simulink model "CACC_konvoy"  (R2026a)
settings: Solver=ode4  StopTime=T_stop  FixedStep=dt
values from neighbouring files (symbols this model uses):
  d0 = 5    [CACC_yonetim.m]
  dt = 0.01    [CACC_yonetim.m]
  ff_u = 1    [CACC_yonetim.m]
  h = 0.6    [CACC_yonetim.m]
  Kd = 0.8    [CACC_yonetim.m]
  Kf = Kf_cacc    (= 0.8)    [CACC_yonetim.m]
  Kp = 0.4    [CACC_yonetim.m]
  L = 4.5    [CACC_yonetim.m]
  p0 = -(1:N) * (d_ss + L)    [CACC_yonetim.m]
  tau = 0.5    [CACC_yonetim.m]
  tauc_max = max(tauc_profil(:, 2)) + dt    [CACC_yonetim.m]
  u_max = 3    [CACC_yonetim.m]
  u_min = -5    [CACC_yonetim.m]
  v0 = 15    [CACC_yonetim.m]
settings Model: Creator=furka  LastModifiedBy=furka

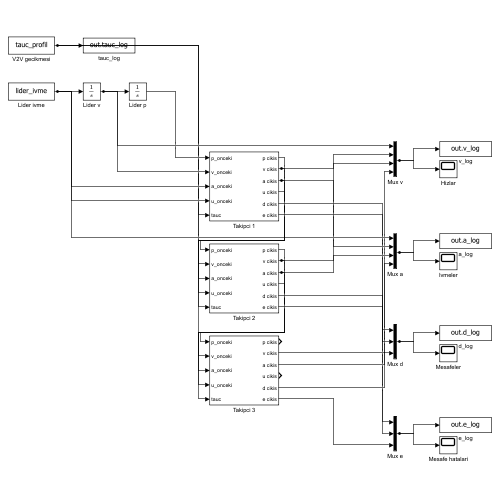
[thumbnail: Simulink's stored preview of the top-level diagram]
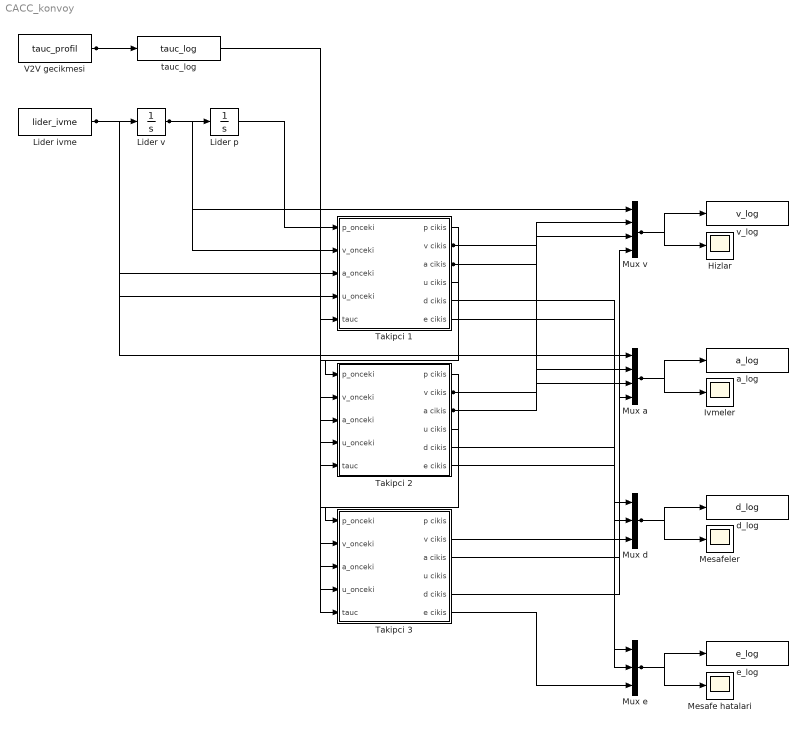
== system CACC_konvoy ==
  Hizlar : Scope
  Ivmeler : Scope
  Lider ivme : FromWorkspace  VariableName=lider_ivme  OutputAfterFinalValue=Holding final value
  Lider p : Integrator
  Lider v : Integrator  InitialCondition=v0
  Mesafe hatalari : Scope
  Mesafeler : Scope
  Mux a : Mux
  Mux d : Mux  Inputs=3
  Mux e : Mux  Inputs=3
  Mux v : Mux
  Takipci 1 : Subsystem
  Takipci 2 : Subsystem
  Takipci 3 : Subsystem
  V2V gecikmesi : FromWorkspace  VariableName=tauc_profil  Interpolate=off  OutputAfterFinalValue=Holding final value
  a_log : ToWorkspace  VariableName=a_log  SampleTime=-1
  d_log : ToWorkspace  VariableName=d_log  SampleTime=-1
  e_log : ToWorkspace  VariableName=e_log  SampleTime=-1
  tauc_log : ToWorkspace  VariableName=tauc_log  SampleTime=-1
  v_log : ToWorkspace  VariableName=v_log  SampleTime=-1
  wires:
  Lider ivme/1 -> Lider v/1, Takipci 1/3(a_onceki), Takipci 1/4(u_onceki), Mux a/1
  Lider v/1 -> Lider p/1, Takipci 1/2(v_onceki), Mux v/1
  Lider p/1 -> Takipci 1/1(p_onceki)
  V2V gecikmesi/1 -> Takipci 1/5(tauc), Takipci 2/5(tauc), Takipci 3/5(tauc), tauc_log/1
  Takipci 1/1(p cikis) -> Takipci 2/1(p_onceki)
  Takipci 1/2(v cikis) -> Takipci 2/2(v_onceki), Mux v/2
  Takipci 1/3(a cikis) -> Takipci 2/3(a_onceki), Mux a/2
  Takipci 1/4(u cikis) -> Takipci 2/4(u_onceki)
  Takipci 2/1(p cikis) -> Takipci 3/1(p_onceki)
  Takipci 2/2(v cikis) -> Takipci 3/2(v_onceki), Mux v/3
  Takipci 2/3(a cikis) -> Takipci 3/3(a_onceki), Mux a/3
  Takipci 2/4(u cikis) -> Takipci 3/4(u_onceki)
  Takipci 3/2(v cikis) -> Mux v/4
  Mux v/1 -> v_log/1, Hizlar/1
  Takipci 3/3(a cikis) -> Mux a/4
  Mux a/1 -> a_log/1, Ivmeler/1
  Takipci 1/5(d cikis) -> Mux d/1
  Takipci 2/5(d cikis) -> Mux d/2
  Takipci 3/5(d cikis) -> Mux d/3
  Mux d/1 -> d_log/1, Mesafeler/1
  Takipci 1/6(e cikis) -> Mux e/1
  Takipci 2/6(e cikis) -> Mux e/2
  Takipci 3/6(e cikis) -> Mux e/3
  Mux e/1 -> e_log/1, Mesafe hatalari/1

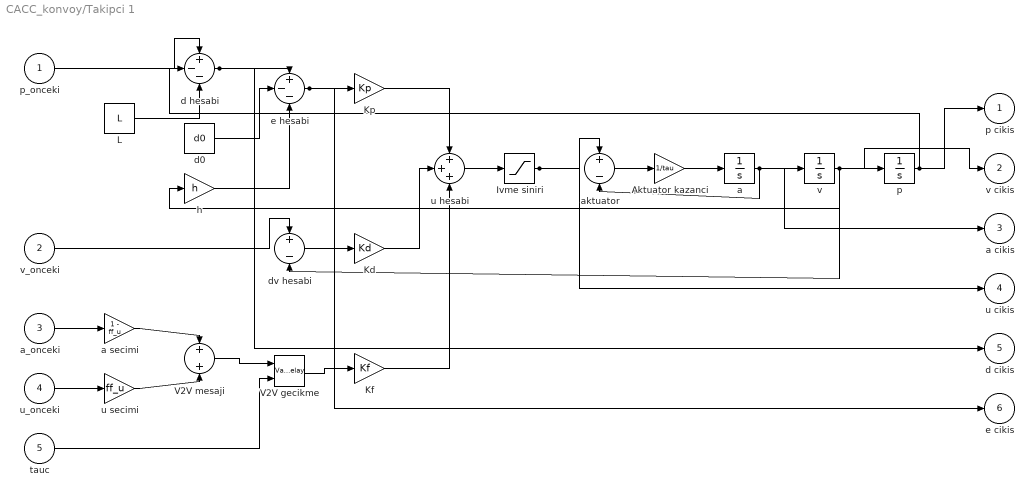
== system CACC_konvoy/Takipci 1 ==
  p_onceki : Inport
  v_onceki : Inport  Port=2
  a_onceki : Inport  Port=3
  u_onceki : Inport  Port=4
  tauc : Inport  Port=5
  Aktuator kazanci : Gain  Gain=1/tau
  Ivme siniri : Saturate  UpperLimit=u_max  LowerLimit=u_min
  Kd : Gain  Gain=Kd
  Kf : Gain  Gain=Kf
  Kp : Gain  Gain=Kp
  L : Constant  Value=L
  V2V gecikme : VariableTransportDelay  MaximumDelay=tauc_max  MaximumPoints=ceil(2*tauc_max/dt) + 100  ZeroDelay=on
  V2V mesaji : Sum
  a : Integrator
  a secimi : Gain  Gain=1 - ff_u
  aktuator : Sum  Inputs=+-
  d hesabi : Sum  Inputs=+--
  d0 : Constant  Value=d0
  dv hesabi : Sum  Inputs=+-
  e hesabi : Sum  Inputs=+--
  h : Gain  Gain=h
  p : Integrator  InitialCondition=p0(1)
  u hesabi : Sum  Inputs=+++
  u secimi : Gain  Gain=ff_u
  v : Integrator  InitialCondition=v0
  p cikis : Outport
  v cikis : Outport  Port=2
  a cikis : Outport  Port=3
  u cikis : Outport  Port=4
  d cikis : Outport  Port=5
  e cikis : Outport  Port=6
  wires:
  p_onceki/1 -> d hesabi/1
  p/1 -> d hesabi/2, p cikis/1
  L/1 -> d hesabi/3
  d hesabi/1 -> e hesabi/1, d cikis/1
  d0/1 -> e hesabi/2
  v/1 -> h/1, dv hesabi/2, p/1, v cikis/1
  h/1 -> e hesabi/3
  v_onceki/1 -> dv hesabi/1
  a_onceki/1 -> a secimi/1
  u_onceki/1 -> u secimi/1
  a secimi/1 -> V2V mesaji/1
  u secimi/1 -> V2V mesaji/2
  V2V mesaji/1 -> V2V gecikme/1
  tauc/1 -> V2V gecikme/2
  V2V gecikme/1 -> Kf/1
  e hesabi/1 -> Kp/1, e cikis/1
  dv hesabi/1 -> Kd/1
  Kp/1 -> u hesabi/1
  Kd/1 -> u hesabi/2
  Kf/1 -> u hesabi/3
  u hesabi/1 -> Ivme siniri/1
  Ivme siniri/1 -> aktuator/1, u cikis/1
  a/1 -> aktuator/2, v/1, a cikis/1
  aktuator/1 -> Aktuator kazanci/1
  Aktuator kazanci/1 -> a/1

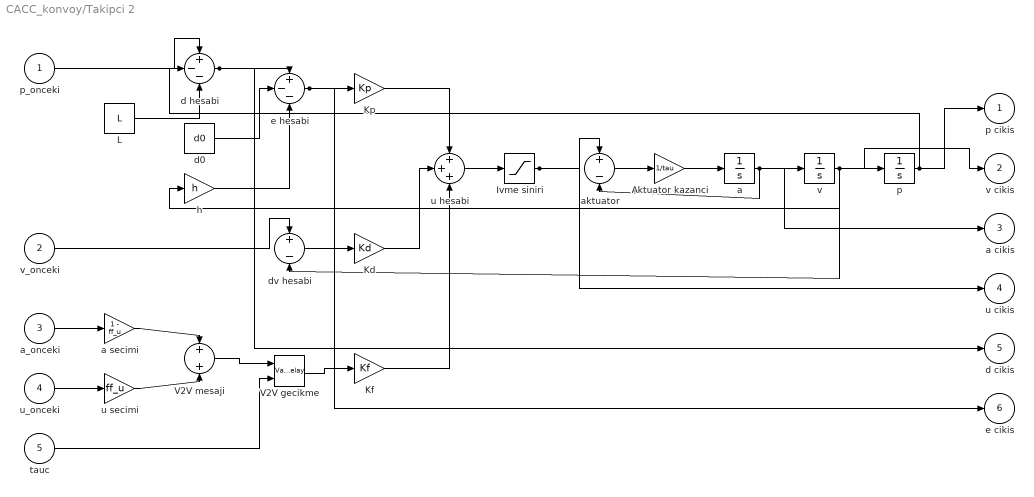
== system CACC_konvoy/Takipci 2 ==
  p_onceki : Inport
  v_onceki : Inport  Port=2
  a_onceki : Inport  Port=3
  u_onceki : Inport  Port=4
  tauc : Inport  Port=5
  Aktuator kazanci : Gain  Gain=1/tau
  Ivme siniri : Saturate  UpperLimit=u_max  LowerLimit=u_min
  Kd : Gain  Gain=Kd
  Kf : Gain  Gain=Kf
  Kp : Gain  Gain=Kp
  L : Constant  Value=L
  V2V gecikme : VariableTransportDelay  MaximumDelay=tauc_max  MaximumPoints=ceil(2*tauc_max/dt) + 100  ZeroDelay=on
  V2V mesaji : Sum
  a : Integrator
  a secimi : Gain  Gain=1 - ff_u
  aktuator : Sum  Inputs=+-
  d hesabi : Sum  Inputs=+--
  d0 : Constant  Value=d0
  dv hesabi : Sum  Inputs=+-
  e hesabi : Sum  Inputs=+--
  h : Gain  Gain=h
  p : Integrator  InitialCondition=p0(2)
  u hesabi : Sum  Inputs=+++
  u secimi : Gain  Gain=ff_u
  v : Integrator  InitialCondition=v0
  p cikis : Outport
  v cikis : Outport  Port=2
  a cikis : Outport  Port=3
  u cikis : Outport  Port=4
  d cikis : Outport  Port=5
  e cikis : Outport  Port=6
  wires:
  p_onceki/1 -> d hesabi/1
  p/1 -> d hesabi/2, p cikis/1
  L/1 -> d hesabi/3
  d hesabi/1 -> e hesabi/1, d cikis/1
  d0/1 -> e hesabi/2
  v/1 -> h/1, dv hesabi/2, p/1, v cikis/1
  h/1 -> e hesabi/3
  v_onceki/1 -> dv hesabi/1
  a_onceki/1 -> a secimi/1
  u_onceki/1 -> u secimi/1
  a secimi/1 -> V2V mesaji/1
  u secimi/1 -> V2V mesaji/2
  V2V mesaji/1 -> V2V gecikme/1
  tauc/1 -> V2V gecikme/2
  V2V gecikme/1 -> Kf/1
  e hesabi/1 -> Kp/1, e cikis/1
  dv hesabi/1 -> Kd/1
  Kp/1 -> u hesabi/1
  Kd/1 -> u hesabi/2
  Kf/1 -> u hesabi/3
  u hesabi/1 -> Ivme siniri/1
  Ivme siniri/1 -> aktuator/1, u cikis/1
  a/1 -> aktuator/2, v/1, a cikis/1
  aktuator/1 -> Aktuator kazanci/1
  Aktuator kazanci/1 -> a/1

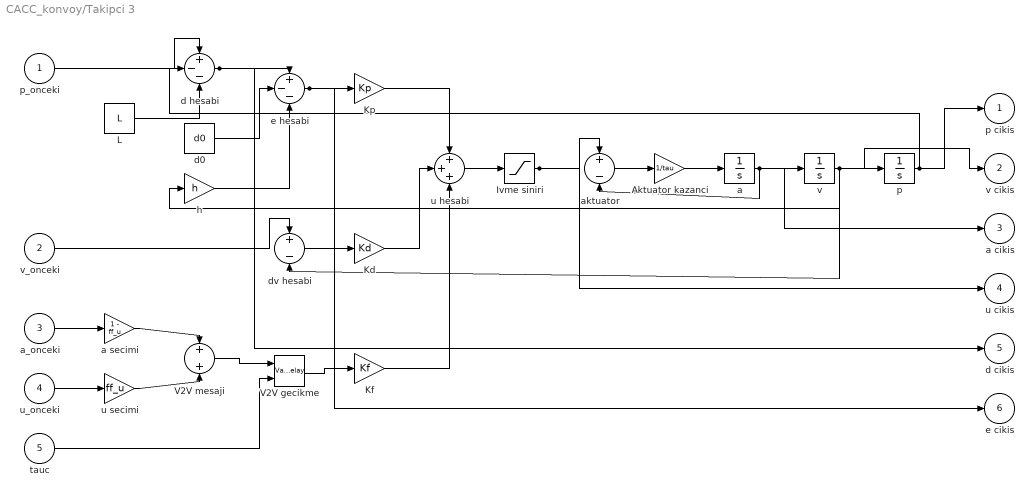
== system CACC_konvoy/Takipci 3 ==
  p_onceki : Inport
  v_onceki : Inport  Port=2
  a_onceki : Inport  Port=3
  u_onceki : Inport  Port=4
  tauc : Inport  Port=5
  Aktuator kazanci : Gain  Gain=1/tau
  Ivme siniri : Saturate  UpperLimit=u_max  LowerLimit=u_min
  Kd : Gain  Gain=Kd
  Kf : Gain  Gain=Kf
  Kp : Gain  Gain=Kp
  L : Constant  Value=L
  V2V gecikme : VariableTransportDelay  MaximumDelay=tauc_max  MaximumPoints=ceil(2*tauc_max/dt) + 100  ZeroDelay=on
  V2V mesaji : Sum
  a : Integrator
  a secimi : Gain  Gain=1 - ff_u
  aktuator : Sum  Inputs=+-
  d hesabi : Sum  Inputs=+--
  d0 : Constant  Value=d0
  dv hesabi : Sum  Inputs=+-
  e hesabi : Sum  Inputs=+--
  h : Gain  Gain=h
  p : Integrator  InitialCondition=p0(3)
  u hesabi : Sum  Inputs=+++
  u secimi : Gain  Gain=ff_u
  v : Integrator  InitialCondition=v0
  p cikis : Outport
  v cikis : Outport  Port=2
  a cikis : Outport  Port=3
  u cikis : Outport  Port=4
  d cikis : Outport  Port=5
  e cikis : Outport  Port=6
  wires:
  p_onceki/1 -> d hesabi/1
  p/1 -> d hesabi/2, p cikis/1
  L/1 -> d hesabi/3
  d hesabi/1 -> e hesabi/1, d cikis/1
  d0/1 -> e hesabi/2
  v/1 -> h/1, dv hesabi/2, p/1, v cikis/1
  h/1 -> e hesabi/3
  v_onceki/1 -> dv hesabi/1
  a_onceki/1 -> a secimi/1
  u_onceki/1 -> u secimi/1
  a secimi/1 -> V2V mesaji/1
  u secimi/1 -> V2V mesaji/2
  V2V mesaji/1 -> V2V gecikme/1
  tauc/1 -> V2V gecikme/2
  V2V gecikme/1 -> Kf/1
  e hesabi/1 -> Kp/1, e cikis/1
  dv hesabi/1 -> Kd/1
  Kp/1 -> u hesabi/1
  Kd/1 -> u hesabi/2
  Kf/1 -> u hesabi/3
  u hesabi/1 -> Ivme siniri/1
  Ivme siniri/1 -> aktuator/1, u cikis/1
  a/1 -> aktuator/2, v/1, a cikis/1
  aktuator/1 -> Aktuator kazanci/1
  Aktuator kazanci/1 -> a/1
